simulink model "UAV_VN1002b"  (Simulink 7.0)
settings: Solver=FixedStepDiscrete  SolverMode=SingleTasking  StartTime=0.0  StopTime=10.0  FixedStep=0.01  RelTol=1e-3
undefined symbols (not defined in the file or in its folder): getImuAcc, Init_onlyOnce, Init_Reset, SPI_VN_init, y1
libraries: dsPICdrivers x9, simulink x1
settings Model: Creator=Dr Wahyudi  LastModifiedBy=Admin
settings OptimizationCC: InlineParams=on  OptimizeModelRefInitCode=on  LifeSpan=1
settings HardwareCC: ProdBitPerInt=16  ProdEndianess=LittleEndian  ProdWordSize=16  ProdHWDeviceType=16-bit Generic
settings RTWCC: SystemTargetFile=dspic.tlc  MakeCommand=make_CreateMPLAB  TemplateMakefile=dspic_pic30_gcc.tmf  PostCodeGenCommand=dsPIC_Compile()  Description=Embedded Target for Microchip dsPIC (real-time)  ProcessScript=dspic_make_rtw_hook
settings RTWCC: CustomSource=|
  | imu.c
  | VN100.c
  | VN_user.c
  | VN_lib.c
  | VN_math.c
settings CodeAppCC: IgnoreCustomStorageClasses=off
settings STFCustomTargetCC: GenFloatMathFcnCalls=ANSI_C  IncludeMdlTerminateFcn=off  CombineOutputUpdateFcns=on  SuppressErrorStatus=on  ERTCustomFileBanners=on  SupportContinuousTime=off  SupportNonInlinedSFcns=off  SystemTargetFile=dspic.tlc
settings ERTTargetCC: GenFloatMathFcnCalls=ANSI_C  CompOptLevelCompliant=off  IncludeMdlTerminateFcn=off  SuppressErrorStatus=on  ModelStepFunctionPrototypeControlCompliant=off  ExtModeMexFile=ext_serial_win32_comm  InlinedParameterPlacement=NonHierarchical  ERTSrcFileBannerTemplate=dsPIC_code_template.cgt  ERTHdrFileBannerTemplate=dsPIC_code_template.cgt  ERTDataSrcFileTemplate=dsPIC_code_template.cgt  ERTDataHdrFileTemplate=dsPIC_code_template.cgt  ERTCustomFileTemplate=dsPIC_main.tlc
settings CustomProperty: DataType=string  Value=C:\PROGRA~1\MATLAB\R2007b\bin\win32\gmake

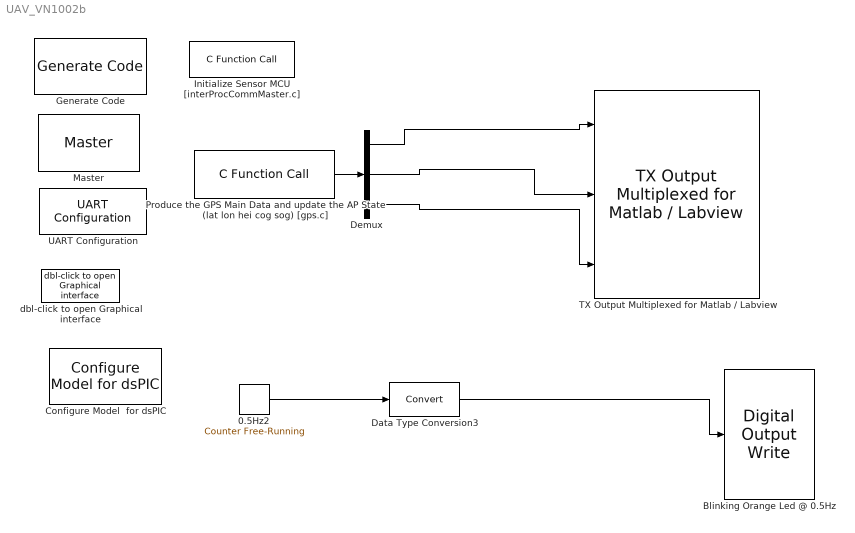
== system UAV_VN1002b ==
  0.5Hz2 : simulink/Sources/Counter Free-Running  SystemSampleTime=-1  NumBits=1  tsamp=1
  Blinking Orange Led @ 0.5Hz : dsPICdrivers/Digital I//O/Digital Output Write  Tag=dsPIC_Digital_Output  Priority=5  PORT=A  Pin=[3]  Simultaneous=off  OrderingInOutPopup=None
  Configure Model  for dsPIC : dsPICdrivers/Simulink Configuration/Configure Model  for dsPIC
  Data Type Conversion3 : DataTypeConversion  OutDataTypeMode=boolean  OutDataType=sfix(16)  OutScaling=2^0
  Demux : Demux  Outputs=3
  Generate Code : dsPICdrivers/Simulink Configuration/Generate Code
  Initialize Sensor MCU [interProcCommMaster.c] : dsPICdrivers/OTHERS/C Function Call  Tag=dsPIC_dsPIC_CFunctionCall  FctUpdate=Output Function  fctName='SPI_VN_init'  INPUT_SIZE=1  INPUT1=--  INPUT2=--  INPUT3=--  OUTPUT_SIZE=1  OUTPUT1=--  SampleTime=inf  InputType=[ ]  OutputType=[ ]  FctDeclaration=extern void SPI_VN_init();  FctCall=SPI_VN_init();  OrderingInOutPopup=None  FctStart=None  FctStart_Name=Init_onlyOnce  FctStart_Declaration=inline extern void Init_onlyOnce();  FctStart_Call=Init_onlyOnce();  FctInit=None  FctInit_Name=Init_Reset  FctInit_Declaration=inline extern void Init_Reset();  FctInit_Call=Init_Reset();
  Master : dsPICdrivers/Master  Tag=dsPIC_MASTER  Priority=1  TimeStepType=Timer1  picType=24fJ128GA010  fcy=16000000  Quartz_33f=8e6  PLLActive_33f=on  fcyDesired_33f=40e6  tmr1="[8  19999  0]"  tmr1Info="Time Step : 0.01  ;   Error : 0%  PR1=19999"  tmr2345="[0  0  0  0]"  tmr2345cfg=[-1 -1 -1 -1]  IOautoConf=on  typePort="[ 10   0   0  10   0   0   0   0   0   0   0   0   0   0   0   0   0   0   0   0   0   0   0   0   0   0   0   0   0   0   0   0   0   0   0   0   0   0   0   0   0   0   0   0   0   0   0   0   0   0   0   0   0   0   0   0   0   0   0   0   0   0   0   0   0   0   0   0   0   0   0   0   0   0   0   0   0   0   0   0   0   0   0   0   4   5   0   0   0   0   0   0   0   0   0   0   0   0   0   0   0   0   0   0   0   0   0   0   0   0   0   0 ]"  TRIS="[ 65526  65535  65535  65535  65535  65535  65535 ]"  ADPCFG=0  MasterBusyPort=None  MasterOverloadPort=None  FOSC=External Clock  ClockSwitchMonitor=Both disabled  TempProtection_33f=TEMP_ON  FPBOR=<empty>  PWRT=64ms  MCLR=<empty>  ICD=ICS_PGD1  JTAGEN=JTAGEN_OFF  PowerSave=off  OverrideFcy=off  NewFcy=1e6  PR2345="[65535  65535  65535  65535]"
  Produce the GPS Main Data and update the AP State (lat lon hei cog sog) [gps.c] : dsPICdrivers/OTHERS/C Function Call  Tag=dsPIC_dsPIC_CFunctionCall  FctUpdate=Output Function  fctName='getImuAcc'  INPUT_SIZE=1  INPUT1=--  INPUT2=--  INPUT3=--  OUTPUT_SIZE=3  OUTPUT1=uint32  SampleTime=.01  InputType=[ ]  OutputType=[ 6 ]  FctDeclaration=extern void getImuAcc(uint32_T* y1);  FctCall=getImuAcc(*%y1);  OrderingInOutPopup=None  FctStart=None  FctStart_Name=Init_onlyOnce  FctStart_Declaration=inline extern void Init_onlyOnce();  FctStart_Call=Init_onlyOnce();  FctInit=None  FctInit_Name=Init_Reset  FctInit_Declaration=inline extern void Init_Reset();  FctInit_Call=Init_Reset();
  TX Output Multiplexed for Matlab / Labview : dsPICdrivers/Serial PORT/TX Output Multiplexed for Matlab // Labview  Tag=dsPIC_TX_Multiplexed  Priority=5  UART=2  CleverSpreadingChk=on  CleverSpreading=1  CHANNEL=[0 1 2]  CHANNELBLOCKED=[]  CHANNELBLOCKED_BITEWISE=0  Status=OK
  UART Configuration : dsPICdrivers/Serial PORT/UART Configuration  Tag=dsPIC_config_UART  Priority=2  UART=2  proposed_BAUD=115200  BAUD=115200  ALT_TX_RX=on  InterruptTxWhen=When Transmit Buffer is empty  TXInterruptPri=1  TxBufferSize=32  TXEN=on  InterruptRxWhen=When Receive Buffer is full (contain 4 characters)  RXInterruptPri=1  RxBufferSize=32  DoNotImplementRxInterrupt=off  DoNotImplementTxInterrupt=off  UxBRG=8  Info="UxBRG = 8   ||  Real Baud : 111111   ||  % error : -3.5494  ||  max 111.1111 Bytes / Step"  RealBaud=0  ERROR=-3.5494  BYTES_STEP=111.1111
  dbl-click to open Graphical interface : dsPICdrivers/Serial PORT/dbl-click to open Graphical interface  Nothing=0
  wires:
  Produce the GPS Main Data and update the AP State (lat lon hei cog sog) [gps.c]/1 -> Demux/1
  Demux/1 -> TX Output Multiplexed for Matlab / Labview/1
  Demux/2 -> TX Output Multiplexed for Matlab / Labview/2
  Demux/3 -> TX Output Multiplexed for Matlab / Labview/3
  0.5Hz2/1 -> Data Type Conversion3/1
  Data Type Conversion3/1 -> Blinking Orange Led @ 0.5Hz/1
